simulink model "Hopper_1DOF"  (R2025a)
settings: Solver=VariableStepAuto  StartTime=0.0  StopTime=50  RelTol=1e-3
values from neighbouring files (symbols this model uses):
  bp = data(:,1)    [load_lookup.m]
  dcg_dMfu_table = [-0.0118909373107 -0.0118767616363 -0.0118626770321 -0.0118486828763 -0.0118347785524 -0.0118209634485 -0.0118072369578 -0.0117935984781 -0.0117800474122 -0.0117665831675 -0.0117532051562 -0.0117399127948 ... (10000 elements, 100x100)]    [cg_I_LUT.mat]    (also in cg_moi_test.m = zeros(length(ox_masses), length(fu_masses)))
  dcg_dMox_table = [-0.0118909373107 0.00235397668616 0.00238701850686 0.00241991378757 0.00245266339356 0.00248526818371 0.00251772901057 0.00255004672045 0.00258222215343 0.00261425614345 0.00264614951832 0.00267790309983 ... (10000 elements, 100x100)]    [cg_I_LUT.mat]    (also in cg_moi_test.m = zeros(length(ox_masses), length(fu_masses)))
  dI_dMfu_table = [0.00516128 0.00516128 0.00516128 0.00516128 0.00516128 0.00516128 0.00516128 0.00516128 0.00516128 0.00516128 0.00516128 0.00516128 ... (90000 elements, 100x100x9)]    [cg_I_LUT.mat]    (also in cg_moi_test.m = zeros(length(ox_masses), length(fu_masses), 9))
  dI_dMox_table = [0.00516128 0.00516128 0.00516128 0.00516128 0.00516128 0.00516128 0.00516128 0.00516128 0.00516128 0.00516128 0.00516128 0.00516128 ... (90000 elements, 100x100x9)]    [cg_I_LUT.mat]    (also in cg_moi_test.m = zeros(length(ox_masses), length(fu_masses), 9))
  fu_masses = [0 0.0909090909091 0.181818181818 0.272727272727 0.363636363636 0.454545454545 0.545454545455 0.636363636364 0.727272727273 0.818181818182 0.909090909091 1 ... (100 elements, 1x100)]    [cg_I_LUT.mat]    (also in cg_moi_test.m = linspace(0,IN.propulsion.fuel_mass,100))
  IN = mission_inputs()    [main.m]
  OUT = Outputs(IN, VEH, TANKS, STRUCT)    [main.m]
  ox_masses = [0 0.161616161616 0.323232323232 0.484848484848 0.646464646465 0.808080808081 0.969696969697 1.13131313131 1.29292929293 1.45454545455 1.61616161616 1.77777777778 ... (100 elements, 1x100)]    [cg_I_LUT.mat]    (also in cg_moi_test.m = linspace(0,IN.propulsion.oxidizer_mass,100))
  tbl1 = data(:,2)    [load_lookup.m]
  tbl2 = data(:,3)    [load_lookup.m]
undefined symbols (not defined in the file or in its folder): cg_init, MoI_init
libraries: dspindex x2, SignalEditorBlockLib x1
settings Model: Creator=asing  LastModifiedBy=asing

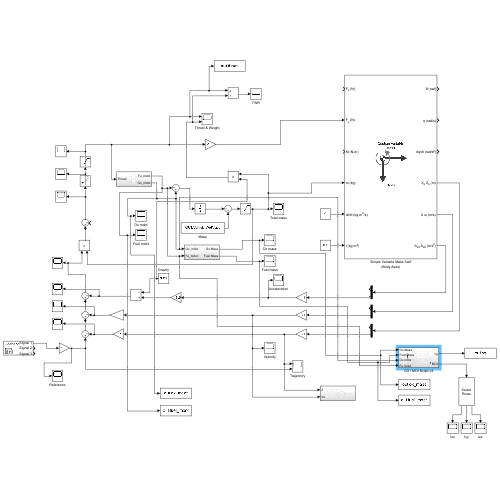
[thumbnail: Simulink's stored preview of the top-level diagram]
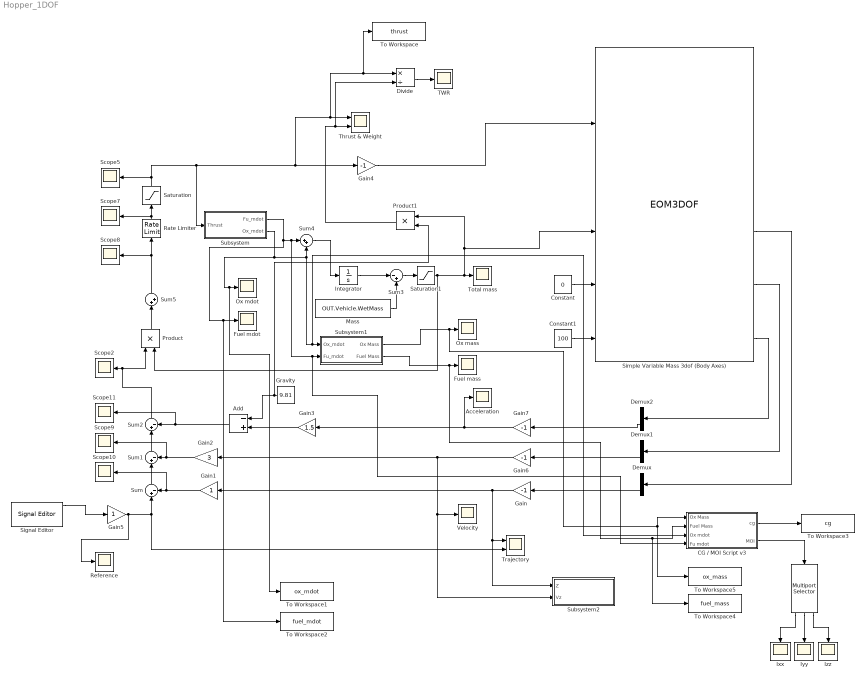
== system Hopper_1DOF ==
  " " : dspindex/Multiport Selector  rowsOrCols=Rows  idxCellArray={1,2,3}  idxErrMode=Clip Index
      settings: LibrarySourceBlock=|
      | dsphdlsupportsigmgmt/Multiport
      | Selector
  Acceleration : Scope
      settings: ActiveDisplayYMinimum=-2.2356377306363511  ActiveDisplayYMaximum=2.9776927592569087  YLabel=Meters per second squared  DataLoggingVariableName=ScopeData3
  Add : Sum  Inputs=-+
  CG / MOI Script v3 : Subsystem
  Constant : Constant  Value=0
  Constant1 : Constant  Value=100
  Demux : Demux  Outputs=2
  Demux1 : Demux  Outputs=2
  Demux2 : Demux  Outputs=2
  Divide : Product  Inputs=*/
  Fuel mass : Scope
      settings: ActiveDisplayYMinimum=4.1848101398701782  ActiveDisplayYMaximum=9.53502109556998  YLabel=Kilograms  DataLoggingVariableName=ScopeData13
  Fuel mdot : Scope
      settings: ActiveDisplayYMinimum=0.13382178992239913  ActiveDisplayYMaximum=0.23326214750133431  YLabel=Kilograms per second  DataLoggingVariableName=ScopeData16
  Gain{,4,6..7} (4 alike) : Gain  Gain=-1
  Gain1 : Gain
  Gain2 : Gain  Gain=3
  Gain3 : Gain  Gain=1.5
  Gain5 : Gain
  Gravity : Constant  Value=9.81
  Integrator : Integrator
  Ixx : Scope
      settings: ActiveDisplayYMinimum=-0.12644047609192863  ActiveDisplayYMaximum=1.1379642848273579  DataLoggingVariableName=ScopeData21
  Iyy : Scope
      settings: ActiveDisplayYMinimum=30.163212884427733  ActiveDisplayYMaximum=49.780093450314517  DataLoggingVariableName=ScopeData26
  Izz : Scope
      settings: ActiveDisplayYMinimum=-2.8210574648941242  ActiveDisplayYMaximum=25.389517184047122  DataLoggingVariableName=ScopeData27
  Mass : Constant  Value=OUT.Vehicle.WetMass
  Ox mass : Scope
      settings: ActiveDisplayYMinimum=6.3696202797403778  ActiveDisplayYMaximum=17.070042191139958  YLabel=Kilograms  DataLoggingVariableName=ScopeData6
  Ox mdot : Scope
      settings: ActiveDisplayYMinimum=-1  ActiveDisplayYMaximum=1  YLabel=Kilograms per second  DataLoggingVariableName=ScopeData15
  Product : Product
  Product1 : Product
  Rate Limiter : RateLimiter  RisingSlewLimit=500  FallingSlewLimit=-500  SampleTimeMode=inherited
  Reference : Scope
      settings: ActiveDisplayYMinimum=-1  ActiveDisplayYMaximum=1  YLabel=Meters  DataLoggingVariableName=ScopeData14
  Saturation : Saturate  UpperLimit=2400  LowerLimit=890  ZeroCross=off
  Saturation1 : Saturate  UpperLimit=OUT.Vehicle.WetMass  LowerLimit=OUT.Vehicle.DryMass
  Scope{2,5,7..11} (7 alike) : Scope
      Scope10 settings: ActiveDisplayYMinimum=2.5668663178756459  ActiveDisplayYMaximum=5.1587087678696406  DataLoggingVariableName=ScopeData10
      Scope11 settings: ActiveDisplayYMinimum=-12.678408094760533  ActiveDisplayYMaximum=11.36813163204156  DataLoggingVariableName=ScopeData11
      Scope2 settings: ActiveDisplayYMinimum=-1.2963468600802761  ActiveDisplayYMaximum=12.866662972523486  DataLoggingVariableName=ScopeData2
      Scope5 settings: ActiveDisplayYMinimum=262.50000000000006  ActiveDisplayYMaximum=2637.5  DataLoggingVariableName=ScopeData5
      Scope7 settings: ActiveDisplayYMinimum=-867.34301243195137  ActiveDisplayYMaximum=3667.8043798582971  DataLoggingVariableName=ScopeData7
      Scope8 settings: ActiveDisplayYMinimum=-820.83409646301129  ActiveDisplayYMaximum=1825.4371218292233  DataLoggingVariableName=ScopeData8
      Scope9 settings: ActiveDisplayYMinimum=-1  ActiveDisplayYMaximum=1  DataLoggingVariableName=ScopeData9
  Signal Editor : SignalEditorBlockLib/Signal Editor  FileName=trajectory_1.mat  ActiveScenario=Scenario  ActiveSignal=Signal 3  IsBus=off  OutputBusObjectStr=Bus: BusObject  SampleTime=0  ZeroCross=off  OutputAfterFinalValue=Setting to zero  Unit=inherit  PreserveSignalName=on  ApplySigPropsToAllScenarios=on  ApplySigPropsToAllSignals=off  SignalPropertySource=Dialog parameters
  Simple Variable Mass 3dof (Body Axes) : EOM3DOF  mtype=Custom Variable  v_ini=0  mass=100  mass_e=50  mass_f=100  Iyy_e=2500  Iyy_f=5000
  Subsystem : Subsystem
  Subsystem1 : Subsystem
  Subsystem2 : Subsystem
  Sum : Sum  Inputs=|+-
  Sum1 : Sum  Inputs=|+-
  Sum2 : Sum  Inputs=|+-
  Sum3 : Sum  Inputs=|-+
  Sum4 : Sum  Inputs=|++
  Sum5 : Sum  Inputs=|++
  TWR : Scope
      settings: ActiveDisplayYMinimum=-1  ActiveDisplayYMaximum=1  DataLoggingVariableName=ScopeData17
  Thrust & Weight : Scope  NumInputPorts=2
      settings: ActiveDisplayYMinimum=828.43747835156955  ActiveDisplayYMaximum=1444.0626948358743  YLabel=Newtons
  To Workspace : ToWorkspace  VariableName=thrust  SaveFormat=Timeseries  SampleTime=-1
  To Workspace1 : ToWorkspace  VariableName=ox_mdot  SaveFormat=Timeseries  SampleTime=-1
  To Workspace2 : ToWorkspace  VariableName=fuel_mdot  SaveFormat=Timeseries  SampleTime=-1
  To Workspace3 : ToWorkspace  VariableName=cg  SaveFormat=Timeseries  SampleTime=-1
  To Workspace4 : ToWorkspace  VariableName=fuel_mass  SaveFormat=Timeseries  SampleTime=-1
  To Workspace5 : ToWorkspace  VariableName=ox_mass  SaveFormat=Timeseries  SampleTime=-1
  Total mass : Scope
      settings: ActiveDisplayYMinimum=104.08322056806487  ActiveDisplayYMaximum=121.9933343110873  DataLoggingVariableName=ScopeData4
  Trajectory : Scope  NumInputPorts=2
      settings: ActiveDisplayYMinimum=-13.443251217870404  ActiveDisplayYMaximum=57.030100710203968  YLabel=Meters
  Velocity : Scope
      settings: ActiveDisplayYMinimum=-4.3862638434935137  ActiveDisplayYMaximum=0.12984319255751209  YLabel=Meters per second  DataLoggingVariableName=ScopeData12
  wires:
  Simple Variable Mass 3dof (Body Axes)/4 -> Demux/1
  Demux/2 -> Gain/1
  Gain/1 -> Subsystem2/1(Z), Trajectory/1, Gain1/1
  Sum/1 -> Sum1/1
  Sum1/1 -> Sum2/1
  Gain1/1 -> Scope10/1, Sum/2
  Simple Variable Mass 3dof (Body Axes)/5 -> Demux1/1
  Simple Variable Mass 3dof (Body Axes)/6 -> Demux2/1
  Demux1/2 -> Gain6/1
  Gain2/1 -> Scope9/1, Sum1/2
  Gain4/1 -> Simple Variable Mass 3dof (Body Axes)/2
  Rate Limiter/1 -> Saturation/1, Scope7/1
  Demux2/2 -> Gain7/1
  Sum4/1 -> Integrator/1
  Integrator/1 -> Sum3/1
  Sum3/1 -> Saturation1/1
  Mass/1 -> Sum3/2
  Sum2/1 -> Product/1, Scope2/1
  Saturation/1 -> Scope5/1, Subsystem/1(Thrust), Gain4/1, To Workspace/1, Divide/1, Thrust & Weight/1
  Gain6/1 -> Subsystem2/2(Vz), Velocity/1, Gain2/1
  Gain7/1 -> Acceleration/1, Gain3/1
  Gain3/1 -> Add/2
  Add/1 -> Scope11/1, Sum2/2
  Constant/1 -> Simple Variable Mass 3dof (Body Axes)/5
  Constant1/1 -> Simple Variable Mass 3dof (Body Axes)/6
  Gravity/1 -> Product1/2, Add/1
  Subsystem/1(Fu_mdot) -> To Workspace2/1, Fuel mdot/1, CG / MOI Script v3/4(Fu mdot), Subsystem1/2(Fu_mdot), Sum4/1
  Subsystem/2(Ox_mdot) -> To Workspace1/1, Ox mdot/1, CG / MOI Script v3/3(Ox mdot), Subsystem1/1(Ox_mdot), Sum4/2
  Subsystem1/1(Ox Mass) -> CG / MOI Script v3/1(Ox Mass), To Workspace5/1, Ox mass/1
  Subsystem1/2(Fuel Mass) -> CG / MOI Script v3/2(Fuel Mass), To Workspace4/1, Fuel mass/1
  Gain5/1 -> Reference/1, Trajectory/2, Sum/1
  Sum5/1 -> Scope8/1, Rate Limiter/1
  Saturation1/1 -> Product/2, Product1/1, Simple Variable Mass 3dof (Body Axes)/4, Total mass/1
  Signal Editor/1 -> Gain5/1
  Product/1 -> Sum5/1
  Product1/1 -> Divide/2, Thrust & Weight/2
  Divide/1 -> TWR/1
  CG / MOI Script v3/1(cg) -> To Workspace3/1
  " "/3 -> Izz/1
  " "/1 -> Ixx/1
  " "/2 -> Iyy/1
  CG / MOI Script v3/2(MOI) -> " "/1

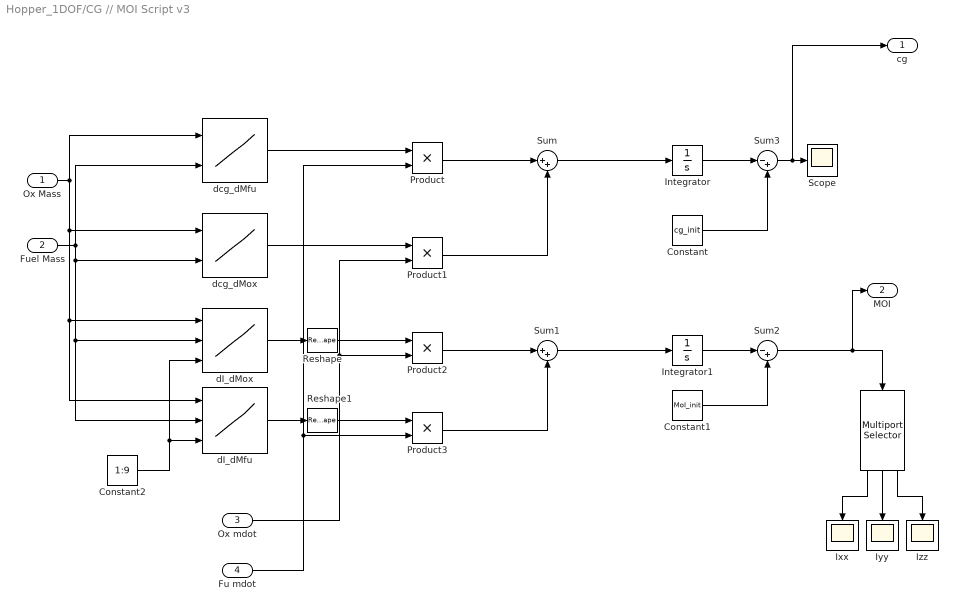
== system Hopper_1DOF/CG // MOI Script v3 ==
  Ox Mass : Inport
  Fuel Mass : Inport  Port=2
  Ox mdot : Inport  Port=3
  Fu mdot : Inport  Port=4
  " " : dspindex/Multiport Selector  rowsOrCols=Rows  idxCellArray={1,2,3}  idxErrMode=Clip Index
      settings: LibrarySourceBlock=|
      | dsphdlsupportsigmgmt/Multiport
      | Selector
  Constant : Constant  Value=cg_init
  Constant1 : Constant  Value=MoI_init
  Constant2 : Constant  Value=1:9
  Integrator : Integrator
  Integrator1 : Integrator
  Ixx : Scope
      settings: ActiveDisplayYMinimum=-0.12644047609192863  ActiveDisplayYMaximum=1.1379642848273579  DataLoggingVariableName=ScopeData19
  Iyy : Scope
      settings: ActiveDisplayYMinimum=30.163212884427733  ActiveDisplayYMaximum=49.780093450314517  DataLoggingVariableName=ScopeData20
  Izz : Scope
      settings: ActiveDisplayYMinimum=-2.8210574648941242  ActiveDisplayYMaximum=25.389517184047122  DataLoggingVariableName=ScopeData22
  Product{,1..3} (4 alike) : Product
  Reshape : Reshape  OutputDimensionality=Customize  OutputDimensions=[3,3]
  Reshape1 : Reshape  OutputDimensionality=Customize  OutputDimensions=[3,3]
  Scope : Scope
      settings: ActiveDisplayYMinimum=1.2968324810484169  ActiveDisplayYMaximum=1.333634125445768  DataLoggingVariableName=ScopeData18
  Sum : Sum  Inputs=|++
  Sum1 : Sum  Inputs=|++
  Sum2 : Sum  Inputs=|-+
  Sum3 : Sum  Inputs=|-+
  dI_dMfu : Lookup_n-D  NumberOfTableDimensions=3  BreakpointsForDimension1=ox_masses  BreakpointsForDimension2=fu_masses  BreakpointsForDimension3=1:9  Table=dI_dMfu_table  InternalRulePriority=Speed  RndMeth=Simplest
      settings: InputPortMap=u0,u1,u2
  dI_dMox : Lookup_n-D  NumberOfTableDimensions=3  BreakpointsForDimension1=ox_masses  BreakpointsForDimension2=fu_masses  BreakpointsForDimension3=1:9  Table=dI_dMox_table  InternalRulePriority=Speed  RndMeth=Simplest
      settings: InputPortMap=u0,u1,u2
  dcg_dMfu : Lookup_n-D  BreakpointsForDimension1=ox_masses  BreakpointsForDimension2=fu_masses  BreakpointsForDimension3=[5, 7]  Table=dcg_dMfu_table  InternalRulePriority=Speed  RndMeth=Simplest
      settings: InputPortMap=u0,u1
  dcg_dMox : Lookup_n-D  BreakpointsForDimension1=ox_masses  BreakpointsForDimension2=fu_masses  BreakpointsForDimension3=[5, 7]  Table=dcg_dMox_table  InternalRulePriority=Speed  RndMeth=Simplest
      settings: InputPortMap=u0,u1
  cg : Outport
  MOI : Outport  Port=2
  wires:
  Ox Mass/1 -> dI_dMfu/1, dI_dMox/1, dcg_dMox/1, dcg_dMfu/1
  Fuel Mass/1 -> dI_dMfu/2, dI_dMox/2, dcg_dMox/2, dcg_dMfu/2
  dcg_dMfu/1 -> Product/1
  Ox mdot/1 -> Product2/2, Product1/2
  dcg_dMox/1 -> Product1/1
  Fu mdot/1 -> Product3/2, Product/2
  dI_dMox/1 -> Reshape/1
  dI_dMfu/1 -> Reshape1/1
  Product/1 -> Sum/1
  Product1/1 -> Sum/2
  Product2/1 -> Sum1/1
  Product3/1 -> Sum1/2
  Sum/1 -> Integrator/1
  Integrator/1 -> Sum3/1
  Constant/1 -> Sum3/2
  Sum3/1 -> cg/1, Scope/1
  Sum1/1 -> Integrator1/1
  Integrator1/1 -> Sum2/1
  Constant1/1 -> Sum2/2
  Reshape/1 -> Product2/1
  Reshape1/1 -> Product3/1
  Constant2/1 -> dI_dMfu/3, dI_dMox/3
  " "/2 -> Iyy/1
  " "/1 -> Ixx/1
  " "/3 -> Izz/1
  Sum2/1 -> MOI/1, " "/1

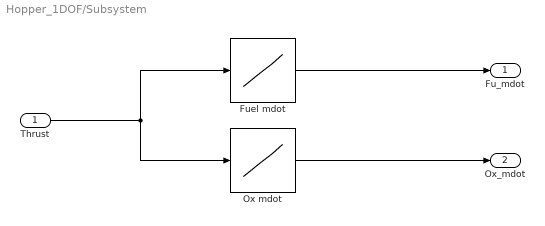
== system Hopper_1DOF/Subsystem ==
  Thrust : Inport
  Fuel mdot : Lookup_n-D  NumberOfTableDimensions=1  BreakpointsForDimension1=bp  Table=tbl2  InternalRulePriority=Speed  RndMeth=Simplest
  Ox mdot : Lookup_n-D  NumberOfTableDimensions=1  BreakpointsForDimension1=bp  Table=tbl1  InternalRulePriority=Speed  RndMeth=Simplest
  Fu_mdot : Outport
  Ox_mdot : Outport  Port=2
  wires:
  Thrust/1 -> Ox mdot/1, Fuel mdot/1
  Fuel mdot/1 -> Fu_mdot/1
  Ox mdot/1 -> Ox_mdot/1

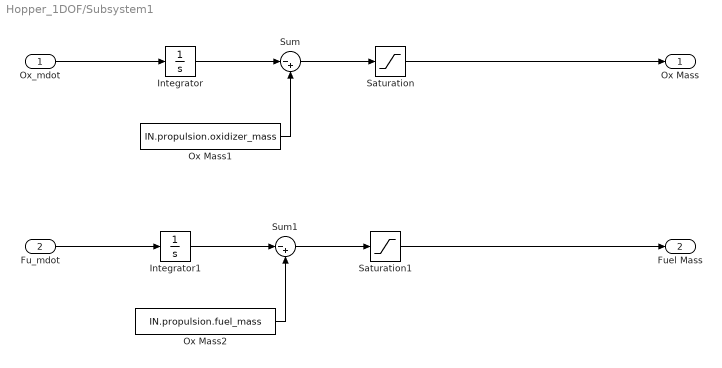
== system Hopper_1DOF/Subsystem1 ==
  Ox_mdot : Inport
  Fu_mdot : Inport  Port=2
  Integrator : Integrator
  Integrator1 : Integrator
  Ox Mass1 : Constant  Value=IN.propulsion.oxidizer_mass
  Ox Mass2 : Constant  Value=IN.propulsion.fuel_mass
  Saturation : Saturate  UpperLimit=IN.propulsion.oxidizer_mass  LowerLimit=0
  Saturation1 : Saturate  UpperLimit=IN.propulsion.fuel_mass  LowerLimit=0
  Sum : Sum  Inputs=|-+
  Sum1 : Sum  Inputs=|-+
  Ox Mass : Outport
  Fuel Mass : Outport  Port=2
  wires:
  Ox_mdot/1 -> Integrator/1
  Integrator/1 -> Sum/1
  Ox Mass1/1 -> Sum/2
  Sum/1 -> Saturation/1
  Saturation/1 -> Ox Mass/1
  Sum1/1 -> Saturation1/1
  Saturation1/1 -> Fuel Mass/1
  Fu_mdot/1 -> Integrator1/1
  Ox Mass2/1 -> Sum1/2
  Integrator1/1 -> Sum1/1

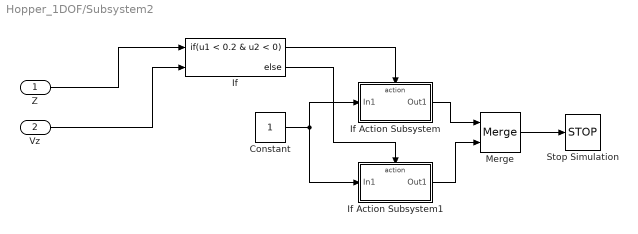
== system Hopper_1DOF/Subsystem2 ==
  Z : Inport
  Vz : Inport  Port=2
  Constant : Constant
  If : If  NumInputs=2  IfExpression=u1 < 0.2 & u2 < 0
  If Action Subsystem : Subsystem  TreatAsAtomicUnit=on
  If Action Subsystem1 : Subsystem  TreatAsAtomicUnit=on
  Merge : Merge
  Stop Simulation : Stop
  wires:
  Z/1 -> If/1
  Vz/1 -> If/2
  If/1 -> If Action Subsystem/Action
  If/2 -> If Action Subsystem1/Action
  Constant/1 -> If Action Subsystem1/1(In1), If Action Subsystem/1(In1)
  If Action Subsystem/1(Out1) -> Merge/1
  If Action Subsystem1/1(Out1) -> Merge/2
  Merge/1 -> Stop Simulation/1

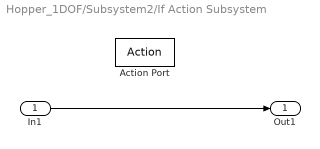
== system Hopper_1DOF/Subsystem2/If Action Subsystem ==
  In1 : Inport
  Action Port : ActionPort  ActionPortLabel=if(u1 < 0.2 & u2 < 0)
  Out1 : Outport
  wires:
  In1/1 -> Out1/1

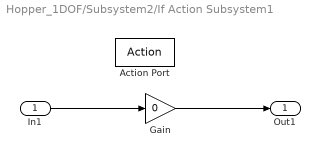
== system Hopper_1DOF/Subsystem2/If Action Subsystem1 ==
  In1 : Inport
  Action Port : ActionPort  ActionPortLabel=else
  Gain : Gain  Gain=0
  Out1 : Outport
  wires:
  In1/1 -> Gain/1
  Gain/1 -> Out1/1
